simulink model "pcm_drl_twin"  (R2026b)
settings: Solver=FixedStepDiscrete  StopTime=31532400  FixedStep=3600
model workspace (MAT data in the model file):
  noise_on = 0
  policy_mode = 0
  wx.time = [0 3600 7200 10800 14400 18000 21600 25200 28800 32400 36000 39600 ... (8760 elements, 8760x1)]
  wx.signals.values = [0 1 2 3 4 5 6 7 8 9 10 11 ... (78840 elements, 8760x9)]
  wx.signals.dimensions = 9
  x0 = [30; 30; 30; 30; 30; 30; 30; 30; 30; 30; 137286.037419; 137286.037419; 137286.037419; 137286.037419; 137286.037419; 137286.037419; 137286.037419; 137286.037419; 137286.037419; 137286.037419; 30; 30; 30; 52; 0; 0; 0.771740525825; 0.0182668616785; 1440; 1]
settings Model: Creator=dudde  LastModifiedBy=dudde
settings DataIOCC: SaveFormat=Array

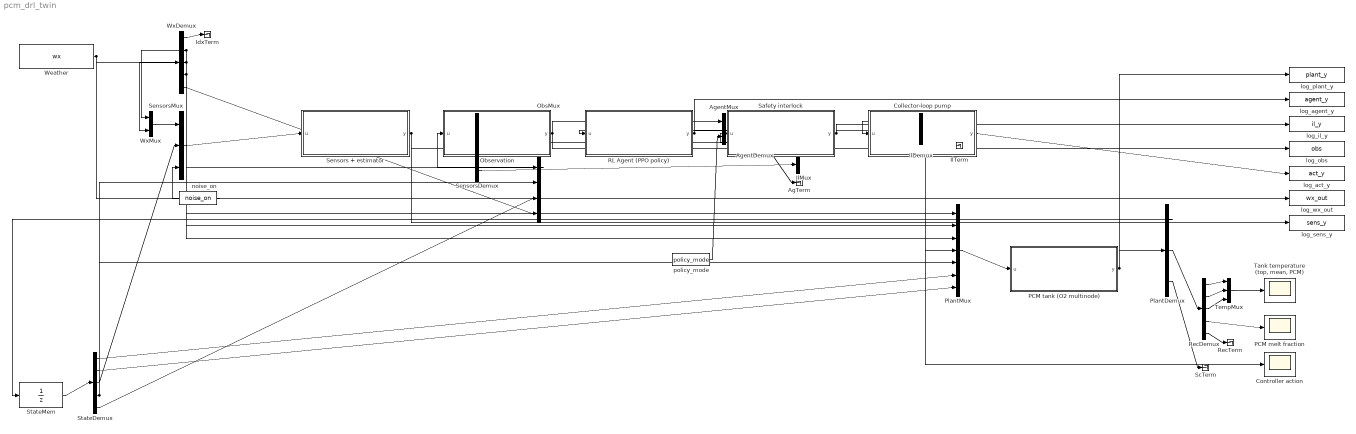
== system pcm_drl_twin ==
  AgTerm : Terminator
  AgentDemux : Demux  Outputs=[1 1]
  AgentMux : Mux  Inputs=2
  Collector-loop pump : MATLAB Function  TreatAsAtomicUnit=on
  Controller action : Scope
  IdxTerm : Terminator
  IlDemux : Demux  Outputs=[1 1]
  IlMux : Mux  Inputs=3
  IlTerm : Terminator
  ObsMux : Mux  Inputs=7
  Observation : MATLAB Function  TreatAsAtomicUnit=on
  PCM melt fraction : Scope
  PCM tank (O2 multinode) : MATLAB Function  TreatAsAtomicUnit=on
  PlantDemux : Demux  Outputs=[30 21 8]
  PlantMux : Mux  Inputs=7
  RL Agent (PPO policy) : MATLAB Function  TreatAsAtomicUnit=on
  RecDemux : Demux  Outputs=[1 1 1 1 17]
  RecTerm : Terminator
  Safety interlock : MATLAB Function  TreatAsAtomicUnit=on
  ScTerm : Terminator
  Sensors + estimator : MATLAB Function  TreatAsAtomicUnit=on
  SensorsDemux : Demux  Outputs=[1 1 8 1]
  SensorsMux : Mux  Inputs=3
  StateDemux : Demux  Outputs=[10 10 8 1 1]
  StateMem : UnitDelay  InitialCondition=x0  SampleTime=3600
  "Tank temperature (top, mean, PCM)" : Scope
  TempMux : Mux  Inputs=3
  Weather : FromWorkspace  VariableName=wx  SampleTime=3600  Interpolate=off  OutputAfterFinalValue=Holding final value
  WxDemux : Demux  Outputs=[1 1 1 1 5]
  WxMux : Mux  Inputs=2
  log_act_y : ToWorkspace  VariableName=act_y  SampleTime=3600
  log_agent_y : ToWorkspace  VariableName=agent_y  SampleTime=3600
  log_il_y : ToWorkspace  VariableName=il_y  SampleTime=3600
  log_obs : ToWorkspace  VariableName=obs  SampleTime=3600
  log_plant_y : ToWorkspace  VariableName=plant_y  SampleTime=3600
  log_sens_y : ToWorkspace  VariableName=sens_y  SampleTime=3600
  log_wx_out : ToWorkspace  VariableName=wx_out  SampleTime=3600
  noise_on : Constant  Value=noise_on  SampleTime=3600
  policy_mode : Constant  Value=policy_mode  SampleTime=3600
  wires:
  Weather/1 -> WxDemux/1, log_wx_out/1
  WxDemux/1 -> IdxTerm/1
  StateMem/1 -> StateDemux/1
  WxDemux/2 -> WxMux/1, PlantMux/1
  WxDemux/3 -> WxMux/2, PlantMux/2
  WxMux/1 -> SensorsMux/1
  StateDemux/3 -> SensorsMux/2
  noise_on/1 -> SensorsMux/3
  SensorsMux/1 -> Sensors + estimator/1(u)
  Sensors + estimator/1(y) -> SensorsDemux/1, log_sens_y/1
  SensorsDemux/3 -> ObsMux/1, IlMux/2
  SensorsDemux/1 -> ObsMux/2
  SensorsDemux/2 -> ObsMux/3
  WxDemux/4 -> ObsMux/4, PlantMux/3
  StateDemux/4 -> ObsMux/5, PlantMux/5
  StateDemux/5 -> ObsMux/6
  WxDemux/5 -> ObsMux/7
  ObsMux/1 -> Observation/1(u)
  Observation/1(y) -> AgentMux/1, log_obs/1
  policy_mode/1 -> AgentMux/2
  AgentMux/1 -> RL Agent (PPO policy)/1(u)
  RL Agent (PPO policy)/1(y) -> AgentDemux/1, log_agent_y/1
  AgentDemux/1 -> IlMux/1
  SensorsDemux/4 -> IlMux/3
  IlMux/1 -> Safety interlock/1(u)
  Safety interlock/1(y) -> IlDemux/1, log_il_y/1
  IlDemux/1 -> Collector-loop pump/1(u), PlantMux/4, Controller action/1
  StateDemux/1 -> PlantMux/6
  StateDemux/2 -> PlantMux/7
  PlantMux/1 -> PCM tank (O2 multinode)/1(u)
  PCM tank (O2 multinode)/1(y) -> PlantDemux/1, log_plant_y/1
  PlantDemux/1 -> StateMem/1
  Collector-loop pump/1(y) -> log_act_y/1
  PlantDemux/2 -> RecDemux/1
  RecDemux/5 -> RecTerm/1
  RecDemux/1 -> TempMux/1
  RecDemux/2 -> TempMux/2
  RecDemux/3 -> TempMux/3
  TempMux/1 -> "Tank temperature (top, mean, PCM)"/1
  RecDemux/4 -> PCM melt fraction/1
  IlDemux/2 -> IlTerm/1
  AgentDemux/2 -> AgTerm/1
  PlantDemux/3 -> ScTerm/1

== matlab function pcm_drl_twin/Sensors + estimator ==
  data: u input size=11; y output size=11
function y = f(u)
[g, ta, r, ok] = sensor_model(u(1), u(2), u(3:10), u(11));
y = [g; ta; r; ok];

== matlab function pcm_drl_twin/RL Agent (PPO policy) ==
  data: u input size=20; y output size=2
function y = f(u)
C = coder.load('twin_consts.mat');
[a, m] = ppo_policy(u(1:19), C.W1, C.b1, C.W2, C.b2, C.Wa, C.ba, u(20));
y = [a; m];

== matlab function pcm_drl_twin/Safety interlock ==
  data: u input size=10; y output size=2
function y = f(u)
C = coder.load('twin_consts.mat');
[a, s] = safety_interlock(u(1), u(2), u(5), u(10), C.P);
y = [a; s];

== matlab function pcm_drl_twin/Collector-loop pump ==
  data: u input size=1; y output size=2
function y = f(u)
y = [double(u == 1); double(u == 0)];

== matlab function pcm_drl_twin/PCM tank (O2 multinode) ==
  data: u input size=25; y output size=59
function y = f(u)
C = coder.load('twin_consts.mat');
K = struct('P', C.P, 'm_w', C.m_w, 'n_caps', C.n_caps, 'loss_ua', C.loss_ua, 'demand24', C.demand24, 'coll', C.coll, 'N', numel(C.m_w));
N = 10;
[T, h, rec, sc] = pcm_plant_hour(u(1), u(2), round(u(3)), u(4), u(6:5+N), u(6+N:5+2*N), K);
ms = u(5);
if rec(10) >= C.draw_thr, ms = 0; else, ms = min(ms + 60, C.min_cap); end
y = [T; h; rec([1 20 2 3 4 10 18 19]); ms; u(4); rec; sc];

== matlab function pcm_drl_twin/Observation ==
  data: u input size=18; y output size=19
function y = f(u)
C = coder.load('twin_consts.mat');
persistent kc
if isempty(kc), kc = 1.0; end
ext4 = zeros(4, 1);
if numel(C.mu) == 19
    [fc, kc] = smart_forecast(u(9), u(14), u(15:17), kc);
    dn = 0; if u(18) >= 0, dn = C.demand24(round(u(18)) + 1); end
    ext4 = [fc; dn];
end
y = double(build_obs(u(1:8), u(9), u(10), round(u(11)), C.P(3), u(12), u(13), C.mu, C.sd, ext4));
